simulink model "EV6_LUT_FourWheel_EV6Battery77p4kWh_PowerCorrected"  (R2024a)
settings: Solver=ode4  StartTime=0  StopTime=60  FixedStep=0.001  RelTol=1e-3
PreLoadFcn:
  | VSS_BICYCLE=Simulink.Variant('Dual=0');
  | VSS_DUAL=Simulink.Variant('Dual=1');
  | Dual=1;
  | load('DriveCycle2.mat')
PostLoadFcn:
  | if any(exist('dsrtsu_mdlpostloadfcn', 'file') ~= 0), dsrtsu_mdlpostloadfcn('Execute', bdroot); end
InitFcn:
  | , if any(exist('rtifpga_mdlclblib', 'file') ~= 0), rtifpga_mdlclblib('Init', bdroot); end,
  | , if any(exist('dsmpb_private', 'file') ~= 0), dsmpb_private('dsmpb_mdlclblib', 'Init', bdroot); end,
  | load('DriveCycle2.mat')
model workspace (MAT data in the model file):
  DiffRatio = 10.65
  EV6_2023_BattBranchCapacity_Ah = 55.5236728838
  EV6_2023_BattEnergy_kWh = 77.4
  EV6_2023_BattNominalVoltage_V = 697
  EV6_2023_BattNumCellsParallel = 2
  EV6_2023_BattNumCellsSeries = 192
  EV6_2023_BattOpenVoltCapBpts = [0 0.1 0.2 0.3 0.4 0.5 0.6 0.7 0.8 0.9 1]
  EV6_2023_BattOpenVoltTbl = [2.96762142548 3.40364281191 3.47417488548 3.54470541822 3.61523441014 3.68576186124 3.75628777151 3.82681214095 3.94527005036 4.07101207308 4.2120755254]
  EV6_2023_BattPackCapacity_Ah = 111.047345768
  EV6_2023_BattResistSocBpts = [0 0.2 0.4 0.6 0.8 1]
  EV6_2023_BattResistTbl = [0.0163620057716 0.0118174152018 0.00807187352333 0.00375663957972 0.00266904525531 0.00103635901355 0.0019014404175 0.0172368903217 0.0121226074867 0.00758541551769 0.00474065349228 0.00337561163613 ... (42 elements, 7x6)]
  EV6_2023_BattResistTempBpts = [243.1 253.1 263.1 273.1 283.1 298.1 313.1]
  EV6_2023_InitialPackOCV_V = 726.471714233
  EV6_2023_InitialSOC = 0.638878863672
  EV6_BattCellCapacity_Ah = 60.3
  EV6_BattInitialSOC = 0.638878863672
  EV6_BattOCV_Cell_V = [2.96762142548 3.40364281191 3.47417488548 3.54470541822 3.61523441014 3.68576186124 3.75628777151 3.82681214095 3.94527005036 4.07101207308 4.2120755254]
  EV6_BattOCV_SOC = [0 0.1 0.2 0.3 0.4 0.5 0.6 0.7 0.8 0.9 1]
  EV6_BattPackCapacity_Ah = 120.6
  EV6_BattParallelCells = 2
  EV6_BattResistanceSOC = [0 0.2 0.4 0.6 0.8 1]
  EV6_BattResistanceTable_Ohm = [0.0163620057716 0.0118174152018 0.00807187352333 0.00375663957972 0.00266904525531 0.00103635901355 0.0019014404175 0.0172368903217 0.0121226074867 0.00758541551769 0.00474065349228 0.00337561163613 ... (42 elements, 7x6)]
  EV6_BattResistanceTemp_K = [243.1 253.1 263.1 273.1 283.1 298.1 313.1]
  EV6_BattSeriesCells = 192
  EV6_FinalDriveRatio = 10.65
  EV6_TargetPackResistance_Ohm = 0.132763804608
  Gas = 0.383333333333
undefined symbols (not defined in the file): accel_bp_mps2, AccelCmd, ActTqLF_Nm_, ActTqLR_Nm_, ActTqRF_Nm_, ActTqRR_Nm_, BattChargeLimitMaxPwr, BattChargeLimitSocBpts, BattChargeLimitTbl, BattDischargeLimitSocBpts, BattDischargeLimitTbl, BattDischargeMaxPwr, BrakeMaxPrs, BrakeMaxTrq, ChassisDistCg2FrontAxle, ChassisDistCg2RearAxle, ChassisVehMass, CltchCmd, CoastDown, DecelCmd, DiscIntNeverNeededParam, EnvGravCnst, EnvPrs, EnvTemp, EV6_RegenTorqueGain, EV6_TractionTorqueGain, front_share_regen_3d, front_share_traction_3d, FuelSpecificGrav, GearCmd, h, InitStates, lgSw, limitedMCT, MCT, MtrEffSpdBpts, MtrEffTbl, MtrEffTrqBpts, MtrPwrMax, MtrTrqMax, out_1, pMCT, RealSimPara, Ref_speed, Ref_time, regen_torque_bp_Nm, speed_bp_kph, SteeringCmd, SupvsryCtrlRegenBrkCutOffTbl, SupvsryCtrlRegenSpdBpts, TestScnrioCycleNum, traction_torque_bp_Nm, US06, VEH
libraries: VSIGenLib x65, simulink x54, etargetslib x38, dsmpblib x24, vehdynlibtire x12, autolibshared x11, vehdynlibsuspension x7, vehdynlibtirecommon x7, autolibpowerinfoutils x6, autolibutils x5, autolibsharedcoupling x4, autolibmappedmotor x4
(part 13 of 19)

== system EV6_LUT_FourWheel_EV6Battery77p4kWh_PowerCorrected/Vehicle Under Test1/Vehicle/Vehicle Dynamics/Vehicle 14DOF/Suspension/MacPherson Front Suspension Solid Axle Rear Suspension/Vehicle Adapter ==
  Veh : Inport
  Bus Creator3 : BusCreator  Inputs=2
  Bus Selector1 : BusSelector  OutputSignals=InertFrm.FrntAxl.Lft.Disp.X,InertFrm.FrntAxl.Lft.Disp.Y,InertFrm.FrntAxl.Lft.Disp.Z,InertFrm.FrntAxl.Rght.Disp.X,InertFrm.FrntAxl.Rght.Disp.Y,InertFrm.FrntAxl.Rght.Disp.Z,InertFrm.RearAxl.Lft.Disp.X,InertFrm.RearAxl.Lft.Disp.Y,InertFrm.RearAxl.Lft.Disp.Z,InertFrm.RearAxl.Rght.Disp.X,InertFrm.RearAxl.Rght.Disp.Y,InertFrm.RearAxl.Rght.Disp.Z
  Bus Selector2 : BusSelector  OutputSignals=BdyFrm.FrntAxl.Lft.Vel.xdot,BdyFrm.FrntAxl.Lft.Vel.ydot,BdyFrm.FrntAxl.Lft.Vel.zdot,BdyFrm.FrntAxl.Rght.Vel.xdot,BdyFrm.FrntAxl.Rght.Vel.ydot,BdyFrm.FrntAxl.Rght.Vel.zdot,BdyFrm.RearAxl.Lft.Vel.xdot,BdyFrm.RearAxl.Lft.Vel.ydot,BdyFrm.RearAxl.Lft.Vel.zdot,BdyFrm.RearAxl.Rght.Vel.xdot,BdyFrm.RearAxl.Rght.Vel.ydot,BdyFrm.RearAxl.Rght.Vel.zdot
  Inertial Frame CG to Axle Offset : Constant  Value=[zeros(2,4);0.434 0.434 0.434 0.434]
  Mux1 : Mux  Inputs=12
  Mux2 : Mux  Inputs=12
  Reshape : Reshape  OutputDimensionality=Customize  OutputDimensions=[3,4]
  Reshape2 : Reshape  OutputDimensionality=Customize  OutputDimensions=[3,4]
  Scope{,1..3} (4 alike) : Scope
  Selector1 : Selector  NumberOfDimensions=2  InputPortWidth=3  IndexOptions=Index vector (dialog),Index vector (dialog)  Indices=[3],[1 2 3 4]  OutputSizes=1,1
  Selector13 : Selector  NumberOfDimensions=2  InputPortWidth=3  IndexOptions=Index vector (dialog),Index vector (dialog)  Indices=[3],[1 2 3 4]  OutputSizes=1,1
  Selector2 : Selector  NumberOfDimensions=2  InputPortWidth=3  IndexOptions=Index vector (dialog),Index vector (dialog)  Indices=[3],[1 2 3 4]  OutputSizes=1,1
  Sum : Sum  Inputs=|+-
  VehSusp : Outport  VectorParamsAs1DForOutWhenUnconnected=off
  wires:
  Sum/1 -> Selector1/1, Bus Creator3/1  "P"
  Inertial Frame CG to Axle Offset/1 -> Sum/2
  Mux2/1 -> Reshape/1
  Mux1/1 -> Reshape2/1
  Bus Selector2/12 -> Mux1/12  "<zdot>"
  Bus Selector2/11 -> Mux1/11  "<ydot>"
  Bus Selector2/10 -> Mux1/10  "<xdot>"
  Bus Selector2/9 -> Mux1/9  "<zdot>"
  Bus Selector2/8 -> Mux1/8  "<ydot>"
  Bus Selector2/7 -> Mux1/7  "<xdot>"
  Bus Selector2/6 -> Mux1/6  "<zdot>"
  Bus Selector2/5 -> Mux1/5  "<ydot>"
  Bus Selector2/4 -> Mux1/4  "<xdot>"
  Bus Selector2/3 -> Mux1/3  "<zdot>"
  Bus Selector2/2 -> Mux1/2  "<ydot>"
  Bus Selector2/1 -> Mux1/1  "<xdot>"
  Bus Selector1/12 -> Mux2/12  "<Z>"
  Bus Selector1/11 -> Mux2/11  "<Y>"
  Bus Selector1/10 -> Mux2/10  "<X>"
  Bus Selector1/9 -> Mux2/9  "<Z>"
  Bus Selector1/8 -> Mux2/8  "<Y>"
  Bus Selector1/7 -> Mux2/7  "<X>"
  Bus Selector1/6 -> Mux2/6  "<Z>"
  Bus Selector1/5 -> Mux2/5  "<Y>"
  Bus Selector1/4 -> Mux2/4  "<X>"
  Bus Selector1/3 -> Mux2/3  "<Z>"
  Bus Selector1/2 -> Mux2/2  "<Y>"
  Bus Selector1/1 -> Mux2/1  "<X>"
  Reshape/1 -> Scope2/1, Selector13/1, Sum/1
  Bus Creator3/1 -> VehSusp/1  "Veh"
  Reshape2/1 -> Selector2/1, Bus Creator3/2  "V"
  Veh/1 -> Bus Selector1/1, Bus Selector2/1
  Selector13/1 -> Scope/1
  Selector1/1 -> Scope1/1
  Selector2/1 -> Scope3/1

== system EV6_LUT_FourWheel_EV6Battery77p4kWh_PowerCorrected/Vehicle Under Test1/Vehicle/Vehicle Dynamics/Vehicle 14DOF/Suspension/MacPherson Front Suspension Solid Axle Rear Suspension/Wheel  Adapter ==
  Wheels : Inport
  Bus Selector : BusSelector  OutputSignals=TireFrame.Fx,TireFrame.Fy
  Bus Selector1 : BusSelector  OutputSignals=TireFrame.Re
  Bus Selector2 : BusSelector  OutputSignals=TireFrame.Mx,TireFrame.My,TireFrame.Mz
  Bus Selector3 : BusSelector  OutputSignals=TireFrame.z,TireFrame.zdot
  Matrix Concatenate : Concatenate  NumInputs=3  Mode=Multidimensional array
  Reshape{,1..7} (8 alike) : Reshape  OutputDimensionality=Row vector (2-D)
  Scope : Scope
  Scope1 : Scope
  Scope2 : Scope
  WhlFx : Outport  VectorParamsAs1DForOutWhenUnconnected=off
  WhlFy : Outport  Port=2  VectorParamsAs1DForOutWhenUnconnected=off
  z : Outport  Port=3  VectorParamsAs1DForOutWhenUnconnected=off
  zdot : Outport  Port=4  VectorParamsAs1DForOutWhenUnconnected=off
  M : Outport  Port=5  VectorParamsAs1DForOutWhenUnconnected=off
  Re : Outport  Port=6  VectorParamsAs1DForOutWhenUnconnected=off
  wires:
  Reshape/1 -> Scope1/1, z/1  "z"
  Matrix Concatenate/1 -> M/1  "M"
  Reshape5/1 -> Matrix Concatenate/3
  Reshape4/1 -> Matrix Concatenate/2
  Reshape3/1 -> Matrix Concatenate/1
  Bus Selector2/3 -> Reshape5/1  "<Mz>"
  Bus Selector2/2 -> Reshape4/1  "<My>"
  Bus Selector2/1 -> Reshape3/1  "<Mx>"
  Reshape1/1 -> Scope/1, Re/1  "Re"
  Bus Selector1/1 -> Reshape1/1  "<Re>"
  Reshape2/1 -> Scope2/1, zdot/1  "zdot"
  Bus Selector3/2 -> Reshape2/1  "<zdot>"
  Wheels/1 -> Bus Selector/1, Bus Selector3/1, Bus Selector2/1, Bus Selector1/1
  Bus Selector3/1 -> Reshape/1  "<z>"
  Bus Selector/2 -> Reshape7/1  "<Fy>"
  Bus Selector/1 -> Reshape6/1  "<Fx>"
  Reshape6/1 -> WhlFx/1
  Reshape7/1 -> WhlFy/1

== system EV6_LUT_FourWheel_EV6Battery77p4kWh_PowerCorrected/Vehicle Under Test1/Vehicle/Vehicle Dynamics/Vehicle 14DOF/Suspension/MacPherson Suspension/Steer Rate Adapter ==
  Veh : Inport
  Add : Sum
  Bus Selector3 : BusSelector  OutputSignals=BdyFrm.Cg.AngVel.r
  Constant : Constant  Value=zeros(1,4)
  Matrix Concatenate : Concatenate  NumInputs=3  Mode=Multidimensional array
  Matrix Concatenate1 : Concatenate  NumInputs=3  Mode=Multidimensional array
  Reshape2 : Reshape  OutputDimensionality=Row vector (2-D)
  Reshape3 : Reshape  OutputDimensionality=Row vector (2-D)
  Reshape4 : Reshape  OutputDimensionality=Row vector (2-D)
  Selector3 : Selector  InputPortWidth=1  IndexOptions=Index vector (dialog)  Indices=[1 1 1 1]  OutputSizes=1
  SteerRates : Constant  Value=zeros(1,4)
  AngVel : Outport  VectorParamsAs1DForOutWhenUnconnected=off
  wires:
  Add/1 -> AngVel/1  "AngVel"
  Veh/1 -> Bus Selector3/1
  Matrix Concatenate1/1 -> Add/1
  Reshape3/1 -> Matrix Concatenate/1, Matrix Concatenate/2
  Reshape4/1 -> Matrix Concatenate/3
  SteerRates/1 -> Reshape2/1
  Matrix Concatenate/1 -> Add/2
  Bus Selector3/1 -> Selector3/1  "<r>"
  Selector3/1 -> Reshape4/1
  Constant/1 -> Reshape3/1
  Reshape2/1 -> Matrix Concatenate1/2, Matrix Concatenate1/3, Matrix Concatenate1/1

== system EV6_LUT_FourWheel_EV6Battery77p4kWh_PowerCorrected/Vehicle Under Test1/Vehicle/Vehicle Dynamics/Vehicle 14DOF/Suspension/MacPherson Suspension/Steering Adapter ==
  Steer : Inport
  Reshape1 : Reshape  OutputDimensionality=Row vector (2-D)
  Selector : Selector  IndexOptions=Index vector (dialog)  Indices=[1 2]  OutputSizes=1
  StrgAng : Outport  VectorParamsAs1DForOutWhenUnconnected=off
  wires:
  Selector/1 -> Reshape1/1
  Steer/1 -> Selector/1
  Reshape1/1 -> StrgAng/1

== system EV6_LUT_FourWheel_EV6Battery77p4kWh_PowerCorrected/Vehicle Under Test1/Vehicle/Vehicle Dynamics/Vehicle 14DOF/Suspension/MacPherson Suspension/Vehicle Adapter ==
  Veh : Inport
  Bus Creator3 : BusCreator  Inputs=2
  Bus Selector1 : BusSelector  OutputSignals=InertFrm.FrntAxl.Lft.Disp.X,InertFrm.FrntAxl.Lft.Disp.Y,InertFrm.FrntAxl.Lft.Disp.Z,InertFrm.FrntAxl.Rght.Disp.X,InertFrm.FrntAxl.Rght.Disp.Y,InertFrm.FrntAxl.Rght.Disp.Z,InertFrm.RearAxl.Lft.Disp.X,InertFrm.RearAxl.Lft.Disp.Y,InertFrm.RearAxl.Lft.Disp.Z,InertFrm.RearAxl.Rght.Disp.X,InertFrm.RearAxl.Rght.Disp.Y,InertFrm.RearAxl.Rght.Disp.Z
  Bus Selector2 : BusSelector  OutputSignals=BdyFrm.FrntAxl.Lft.Vel.xdot,BdyFrm.FrntAxl.Lft.Vel.ydot,BdyFrm.FrntAxl.Lft.Vel.zdot,BdyFrm.FrntAxl.Rght.Vel.xdot,BdyFrm.FrntAxl.Rght.Vel.ydot,BdyFrm.FrntAxl.Rght.Vel.zdot,BdyFrm.RearAxl.Lft.Vel.xdot,BdyFrm.RearAxl.Lft.Vel.ydot,BdyFrm.RearAxl.Lft.Vel.zdot,BdyFrm.RearAxl.Rght.Vel.xdot,BdyFrm.RearAxl.Rght.Vel.ydot,BdyFrm.RearAxl.Rght.Vel.zdot
  Inertial Frame CG to Axle Offset : Constant  Value=[zeros(2,4);h*ones(1,4)]
  Mux1 : Mux  Inputs=12
  Mux2 : Mux  Inputs=12
  Reshape1 : Reshape  OutputDimensionality=Customize  OutputDimensions=[3,4]
  Reshape2 : Reshape  OutputDimensionality=Customize  OutputDimensions=[3,4]
  Sum : Sum  Inputs=|+-
  VehSusp : Outport  VectorParamsAs1DForOutWhenUnconnected=off
  wires:
  Reshape1/1 -> Sum/1
  Mux2/1 -> Reshape1/1
  Veh/1 -> Bus Selector1/1, Bus Selector2/1
  Sum/1 -> Bus Creator3/1  "P"
  Inertial Frame CG to Axle Offset/1 -> Sum/2
  Mux1/1 -> Reshape2/1
  Bus Selector2/12 -> Mux1/12  "<zdot>"
  Bus Selector2/11 -> Mux1/11  "<ydot>"
  Bus Selector2/10 -> Mux1/10  "<xdot>"
  Bus Selector2/9 -> Mux1/9  "<zdot>"
  Bus Selector2/8 -> Mux1/8  "<ydot>"
  Bus Selector2/7 -> Mux1/7  "<xdot>"
  Bus Selector2/6 -> Mux1/6  "<zdot>"
  Bus Selector2/5 -> Mux1/5  "<ydot>"
  Bus Selector2/4 -> Mux1/4  "<xdot>"
  Bus Selector2/3 -> Mux1/3  "<zdot>"
  Bus Selector2/2 -> Mux1/2  "<ydot>"
  Bus Selector2/1 -> Mux1/1  "<xdot>"
  Bus Selector1/12 -> Mux2/12  "<Z>"
  Bus Selector1/11 -> Mux2/11  "<Y>"
  Bus Selector1/10 -> Mux2/10  "<X>"
  Bus Selector1/9 -> Mux2/9  "<Z>"
  Bus Selector1/8 -> Mux2/8  "<Y>"
  Bus Selector1/7 -> Mux2/7  "<X>"
  Bus Selector1/6 -> Mux2/6  "<Z>"
  Bus Selector1/5 -> Mux2/5  "<Y>"
  Bus Selector1/4 -> Mux2/4  "<X>"
  Bus Selector1/3 -> Mux2/3  "<Z>"
  Bus Selector1/2 -> Mux2/2  "<Y>"
  Bus Selector1/1 -> Mux2/1  "<X>"
  Bus Creator3/1 -> VehSusp/1  "Veh"
  Reshape2/1 -> Bus Creator3/2  "V"

== system EV6_LUT_FourWheel_EV6Battery77p4kWh_PowerCorrected/Vehicle Under Test1/Vehicle/Vehicle Dynamics/Vehicle 14DOF/Suspension/MacPherson Suspension/Wheel  Adapter ==
  Wheels : Inport
  Bus Selector : BusSelector  OutputSignals=TireFrame.Fx,TireFrame.Fy
  Bus Selector1 : BusSelector  OutputSignals=TireFrame.Re
  Bus Selector2 : BusSelector  OutputSignals=TireFrame.Mx,TireFrame.My,TireFrame.Mz
  Bus Selector3 : BusSelector  OutputSignals=TireFrame.z,TireFrame.zdot
  Matrix Concatenate : Concatenate  NumInputs=3  Mode=Multidimensional array
  Reshape{,1..7} (8 alike) : Reshape  OutputDimensionality=Row vector (2-D)
  WhlFx : Outport  VectorParamsAs1DForOutWhenUnconnected=off
  WhlFy : Outport  Port=2  VectorParamsAs1DForOutWhenUnconnected=off
  z : Outport  Port=3  VectorParamsAs1DForOutWhenUnconnected=off
  zdot : Outport  Port=4  VectorParamsAs1DForOutWhenUnconnected=off
  M : Outport  Port=5  VectorParamsAs1DForOutWhenUnconnected=off
  Re : Outport  Port=6  VectorParamsAs1DForOutWhenUnconnected=off
  wires:
  Reshape/1 -> z/1  "z"
  Matrix Concatenate/1 -> M/1  "M"
  Reshape5/1 -> Matrix Concatenate/3
  Reshape4/1 -> Matrix Concatenate/2
  Reshape3/1 -> Matrix Concatenate/1
  Bus Selector2/3 -> Reshape5/1  "<Mz>"
  Bus Selector2/2 -> Reshape4/1  "<My>"
  Bus Selector2/1 -> Reshape3/1  "<Mx>"
  Reshape1/1 -> Re/1  "Re"
  Bus Selector1/1 -> Reshape1/1  "<Re>"
  Reshape2/1 -> zdot/1  "zdot"
  Bus Selector3/2 -> Reshape2/1  "<zdot>"
  Wheels/1 -> Bus Selector/1, Bus Selector3/1, Bus Selector2/1, Bus Selector1/1
  Bus Selector3/1 -> Reshape/1  "<z>"
  Bus Selector/2 -> Reshape7/1  "<Fy>"
  Bus Selector/1 -> Reshape6/1  "<Fx>"
  Reshape6/1 -> WhlFx/1
  Reshape7/1 -> WhlFy/1

== system EV6_LUT_FourWheel_EV6Battery77p4kWh_PowerCorrected/Vehicle Under Test1/Vehicle/Vehicle Dynamics/Vehicle 14DOF/Suspension/Mapped Suspension/Steer Rate Adapter ==
  Veh : Inport
  Add : Sum
  Bus Selector3 : BusSelector  OutputSignals=BdyFrm.Cg.AngVel.r
  Constant : Constant  Value=zeros(1,4)
  Matrix Concatenate : Concatenate  NumInputs=3  Mode=Multidimensional array
  Matrix Concatenate1 : Concatenate  NumInputs=3  Mode=Multidimensional array
  Reshape2 : Reshape  OutputDimensionality=Row vector (2-D)
  Reshape3 : Reshape  OutputDimensionality=Row vector (2-D)
  Reshape4 : Reshape  OutputDimensionality=Row vector (2-D)
  Selector3 : Selector  InputPortWidth=1  IndexOptions=Index vector (dialog)  Indices=[1 1 1 1]  OutputSizes=1
  SteerRates : Constant  Value=zeros(1,4)
  AngVel : Outport  VectorParamsAs1DForOutWhenUnconnected=off
  wires:
  Add/1 -> AngVel/1  "AngVel"
  Veh/1 -> Bus Selector3/1
  Matrix Concatenate1/1 -> Add/1
  Reshape3/1 -> Matrix Concatenate/1, Matrix Concatenate/2
  Reshape4/1 -> Matrix Concatenate/3
  SteerRates/1 -> Reshape2/1
  Matrix Concatenate/1 -> Add/2
  Bus Selector3/1 -> Selector3/1  "<r>"
  Selector3/1 -> Reshape4/1
  Constant/1 -> Reshape3/1
  Reshape2/1 -> Matrix Concatenate1/2, Matrix Concatenate1/3, Matrix Concatenate1/1

== system EV6_LUT_FourWheel_EV6Battery77p4kWh_PowerCorrected/Vehicle Under Test1/Vehicle/Vehicle Dynamics/Vehicle 14DOF/Suspension/Mapped Suspension/Vehicle Adapter ==
  Veh : Inport
  Bus Creator3 : BusCreator  Inputs=2
  Bus Selector1 : BusSelector  OutputSignals=InertFrm.FrntAxl.Lft.Disp.X,InertFrm.FrntAxl.Lft.Disp.Y,InertFrm.FrntAxl.Lft.Disp.Z,InertFrm.FrntAxl.Rght.Disp.X,InertFrm.FrntAxl.Rght.Disp.Y,InertFrm.FrntAxl.Rght.Disp.Z,InertFrm.RearAxl.Lft.Disp.X,InertFrm.RearAxl.Lft.Disp.Y,InertFrm.RearAxl.Lft.Disp.Z,InertFrm.RearAxl.Rght.Disp.X,InertFrm.RearAxl.Rght.Disp.Y,InertFrm.RearAxl.Rght.Disp.Z
  Bus Selector2 : BusSelector  OutputSignals=BdyFrm.FrntAxl.Lft.Vel.xdot,BdyFrm.FrntAxl.Lft.Vel.ydot,BdyFrm.FrntAxl.Lft.Vel.zdot,BdyFrm.FrntAxl.Rght.Vel.xdot,BdyFrm.FrntAxl.Rght.Vel.ydot,BdyFrm.FrntAxl.Rght.Vel.zdot,BdyFrm.RearAxl.Lft.Vel.xdot,BdyFrm.RearAxl.Lft.Vel.ydot,BdyFrm.RearAxl.Lft.Vel.zdot,BdyFrm.RearAxl.Rght.Vel.xdot,BdyFrm.RearAxl.Rght.Vel.ydot,BdyFrm.RearAxl.Rght.Vel.zdot
  Inertial Frame CG to Axle Offset : Constant  Value=[zeros(2,4);h*ones(1,4)]
  Mux1 : Mux  Inputs=12
  Mux2 : Mux  Inputs=12
  Reshape : Reshape  OutputDimensionality=Customize  OutputDimensions=[3,4]
  Reshape2 : Reshape  OutputDimensionality=Customize  OutputDimensions=[3,4]
  Sum : Sum  Inputs=|+-
  VehSusp : Outport  VectorParamsAs1DForOutWhenUnconnected=off
  wires:
  Sum/1 -> Bus Creator3/1  "P"
  Inertial Frame CG to Axle Offset/1 -> Sum/2
  Mux2/1 -> Reshape/1
  Mux1/1 -> Reshape2/1
  Bus Selector2/12 -> Mux1/12  "<zdot>"
  Bus Selector2/11 -> Mux1/11  "<ydot>"
  Bus Selector2/10 -> Mux1/10  "<xdot>"
  Bus Selector2/9 -> Mux1/9  "<zdot>"
  Bus Selector2/8 -> Mux1/8  "<ydot>"
  Bus Selector2/7 -> Mux1/7  "<xdot>"
  Bus Selector2/6 -> Mux1/6  "<zdot>"
  Bus Selector2/5 -> Mux1/5  "<ydot>"
  Bus Selector2/4 -> Mux1/4  "<xdot>"
  Bus Selector2/3 -> Mux1/3  "<zdot>"
  Bus Selector2/2 -> Mux1/2  "<ydot>"
  Bus Selector2/1 -> Mux1/1  "<xdot>"
  Bus Selector1/12 -> Mux2/12  "<Z>"
  Bus Selector1/11 -> Mux2/11  "<Y>"
  Bus Selector1/10 -> Mux2/10  "<X>"
  Bus Selector1/9 -> Mux2/9  "<Z>"
  Bus Selector1/8 -> Mux2/8  "<Y>"
  Bus Selector1/7 -> Mux2/7  "<X>"
  Bus Selector1/6 -> Mux2/6  "<Z>"
  Bus Selector1/5 -> Mux2/5  "<Y>"
  Bus Selector1/4 -> Mux2/4  "<X>"
  Bus Selector1/3 -> Mux2/3  "<Z>"
  Bus Selector1/2 -> Mux2/2  "<Y>"
  Bus Selector1/1 -> Mux2/1  "<X>"
  Reshape/1 -> Sum/1
  Bus Creator3/1 -> VehSusp/1  "Veh"
  Reshape2/1 -> Bus Creator3/2  "V"
  Veh/1 -> Bus Selector1/1, Bus Selector2/1

== system EV6_LUT_FourWheel_EV6Battery77p4kWh_PowerCorrected/Vehicle Under Test1/Vehicle/Vehicle Dynamics/Vehicle 14DOF/Suspension/Mapped Suspension/Wheel  Adapter ==
  Wheels : Inport
  Bus Selector : BusSelector  OutputSignals=TireFrame.Fx,TireFrame.Fy
  Bus Selector1 : BusSelector  OutputSignals=TireFrame.Re
  Bus Selector2 : BusSelector  OutputSignals=TireFrame.Mx,TireFrame.My,TireFrame.Mz
  Bus Selector3 : BusSelector  OutputSignals=TireFrame.z,TireFrame.zdot
  Matrix Concatenate : Concatenate  NumInputs=3  Mode=Multidimensional array
  Reshape{,1..7} (8 alike) : Reshape  OutputDimensionality=Row vector (2-D)
  WhlFx : Outport  VectorParamsAs1DForOutWhenUnconnected=off
  WhlFy : Outport  Port=2  VectorParamsAs1DForOutWhenUnconnected=off
  z : Outport  Port=3  VectorParamsAs1DForOutWhenUnconnected=off
  zdot : Outport  Port=4  VectorParamsAs1DForOutWhenUnconnected=off
  M : Outport  Port=5  VectorParamsAs1DForOutWhenUnconnected=off
  Re : Outport  Port=6  VectorParamsAs1DForOutWhenUnconnected=off
  wires:
  Reshape/1 -> z/1  "z"
  Matrix Concatenate/1 -> M/1  "M"
  Reshape5/1 -> Matrix Concatenate/3
  Reshape4/1 -> Matrix Concatenate/2
  Reshape3/1 -> Matrix Concatenate/1
  Bus Selector2/3 -> Reshape5/1  "<Mz>"
  Bus Selector2/2 -> Reshape4/1  "<My>"
  Bus Selector2/1 -> Reshape3/1  "<Mx>"
  Reshape1/1 -> Re/1  "Re"
  Bus Selector1/1 -> Reshape1/1  "<Re>"
  Reshape2/1 -> zdot/1  "zdot"
  Bus Selector3/2 -> Reshape2/1  "<zdot>"
  Wheels/1 -> Bus Selector/1, Bus Selector3/1, Bus Selector2/1, Bus Selector1/1
  Bus Selector3/1 -> Reshape/1  "<z>"
  Bus Selector/2 -> Reshape7/1  "<Fy>"
  Bus Selector/1 -> Reshape6/1  "<Fx>"
  Reshape6/1 -> WhlFx/1
  Reshape7/1 -> WhlFy/1

== system EV6_LUT_FourWheel_EV6Battery77p4kWh_PowerCorrected/Vehicle Under Test1/Vehicle/Vehicle Dynamics/Vehicle 14DOF/Vehicle/Variant Subsystem/3DOF ==
  Suspension : Inport
  Wind : Inport  Port=2
  Bus Selector1 : BusSelector  OutputSignals=Veh.F
  Permute Dimensions : PermuteDimensions
  Permute Dimensions1 : PermuteDimensions
  Scope : Scope
  Scope1 : Scope  NumInputPorts=2
  Scope2 : Scope  NumInputPorts=2
  Scope3 : Scope
  Scope4 : Scope
  Selector : Selector  NumberOfDimensions=2  InputPortWidth=3  IndexOptions=Index vector (dialog),Index vector (dialog)  Indices=[1 2],[1 2]  OutputSizes=1,1
  Selector1 : Selector  NumberOfDimensions=2  InputPortWidth=3  IndexOptions=Index vector (dialog),Index vector (dialog)  Indices=[1 2],[3 4]  OutputSizes=1,1
  Signal Specification : SignalSpecification  Unit=N
  Signal Specification1 : SignalSpecification  Unit=N
  Terminator{,1..5} (6 alike) : Terminator
  Vehicle Body 3DOF Dual Track : autolibshared/Vehicle Body 3DOF Single Track  trackMode=Dual  inputMode=External forces  frontSteerMode=off  rearSteerMode=off  windMode=on  muMode=off  extFMode=off  extMMode=off  htchFMode=off  htchMMode=off  extXo=off  extpsio=off  extxdoto=off  extro=off  extYo=off  extTamb=off  extydoto=off  aMode=2  NF=2  NR=2  m=2040  a=1.4  b=1.6  h=0.5  dh=1  hh=0.2  X_o=0  xdot_o=0  CalphaMode=off  sigmaMode=on  d=0  hl=0  w=1.9.*[1 1]  Cy_f=12e3  Cy_r=11e3  sigma_f=.1  sigma_r=.1  alpha_f_brk=[-.1 .1]  Cy_f_data=[-9e3 9e3]  alpha_r_brk=[-.1 .1]  Cy_r_data=[-9e3 9e3]  Y_o=0  ydot_o=0  Izz=2100  psi_o=0  r_o=0  Af=2  Cd=.3  Cl=.1  Cpm=.1  beta_w=[0:0.001:0.01]  Cs=[0:0.01:0.1]  Cym=[0:0.001:0.01]  Pabs=101325  Tair=273  g=9.81  mu=1  xdot_tol=.1  Fznom=5000  Fxtire_sat=7e5  Fytire_sat=7e5  longOff=0  latOff=0  vertOff=0  wrapAng=on
  VehFdbk : Outport  VectorParamsAs1DForOutWhenUnconnected=off
  wires:
  Wind/1 -> Vehicle Body 3DOF Dual Track/3
  Permute Dimensions/1 -> Signal Specification1/1
  Permute Dimensions1/1 -> Signal Specification/1
  Vehicle Body 3DOF Dual Track/7 -> Terminator5/1, Scope1/2
  Vehicle Body 3DOF Dual Track/1 -> VehFdbk/1
  Vehicle Body 3DOF Dual Track/2 -> Terminator/1, Scope/1
  Vehicle Body 3DOF Dual Track/4 -> Terminator2/1
  Vehicle Body 3DOF Dual Track/6 -> Terminator4/1, Scope1/1
  Signal Specification/1 -> Scope4/1, Vehicle Body 3DOF Dual Track/2
  Vehicle Body 3DOF Dual Track/3 -> Terminator1/1
  Signal Specification1/1 -> Vehicle Body 3DOF Dual Track/1, Scope3/1
  Vehicle Body 3DOF Dual Track/5 -> Terminator3/1
  Suspension/1 -> Bus Selector1/1
  Selector1/1 -> Permute Dimensions1/1
  Selector/1 -> Permute Dimensions/1
  Bus Selector1/1 -> Selector/1, Selector1/1  "<F>"

== system EV6_LUT_FourWheel_EV6Battery77p4kWh_PowerCorrected/Vehicle Under Test1/Vehicle/Vehicle Dynamics/Vehicle 14DOF/Vehicle/Variant Subsystem/6DOF ==
  Suspension : Inport
  Wind : Inport  Port=2
  Bus Selector3 : BusSelector  OutputSignals=Veh.F,Veh.M
  Constant : Constant  Value=[0;0;0]
  Constant1 : Constant  Value=[0;0;0]
  Terminator{,1..5} (6 alike) : Terminator
  Vehicle Body 6DOF : vehdynlibeom/Vehicle Body 6DOF  extPos=on  extVel=on  extEuler=on  extRotRate=on  htchFMode=off  htchMMode=off  m=2040  a=1.4  b=1.6  d=0  h=0.5  dh=1  hl=0  hh=0.1  Xe_o=[0,0,0.1]  xbdot_o=[0,0,0]  eul_o=[0,0,0]  p_o=[0,0,0]  Iveh=[430 0 0; 0 1900 0; 0 0 2100]  w=[1.9,1.9]  z1m=0  z1R=[-.25,.125,.15]  z1I=[1.4,-.2,.1;-.2,1.4,.1;.1,.1,2.25].*0  z2m=0  z2R=[1.4,0,.8]  z2I=[1.4,-.2,.1;-.2,1.4,.1;.1,.1,2.25].*0  z3m=0  z3R=[.75,-.5,.4]  z3I=[5,-.1,-2;-2,9,.1;-.1,.1,6].*0  z4m=0  z4R=[.75,.5,.4]  z4I=[5,-.1,-2;-2,9,.1;-.1,.1,6].*0  z5m=0  z5R=[1.25,-.5,.4]  z5I=[5,-.1,-2;-2,9,.1;-.1,.1,6].*0  z6m=0  z6R=[1.25,-.5,.4]  z6I=[5,-.1,-2;-2,9,.1;-.1,.1,6].*0  z7m=0  z7R=[2,0,.25]  z7I=[1.4,-.2,.1;-.2,1.4,.1;.1,.1,2.25].*0  Af=2  Cd=.3  Cl=.1  Cpm=.1  beta_w=[0:0.001:0.01]  Cs=[0:0.01:0.1]  Cym=[0:0.001:0.01]  Pabs=101325  extTamb=off  Tair=273  g=9.81  xdot_tol=.1  longOff=0  latOff=0  vertOff=0  wrapAng=on  aMode=2
  VehFdbk : Outport  VectorParamsAs1DForOutWhenUnconnected=off
  wires:
  Vehicle Body 6DOF/7 -> Terminator5/1
  Vehicle Body 6DOF/6 -> Terminator4/1
  Vehicle Body 6DOF/5 -> Terminator3/1
  Vehicle Body 6DOF/4 -> Terminator2/1
  Vehicle Body 6DOF/3 -> Terminator1/1
  Vehicle Body 6DOF/2 -> Terminator/1
  Constant1/1 -> Vehicle Body 6DOF/4
  Vehicle Body 6DOF/1 -> VehFdbk/1  "VehFdbk"
  Suspension/1 -> Bus Selector3/1
  Constant/1 -> Vehicle Body 6DOF/3
  Wind/1 -> Vehicle Body 6DOF/5
  Bus Selector3/1 -> Vehicle Body 6DOF/1  "<F>"
  Bus Selector3/2 -> Vehicle Body 6DOF/2  "<M>"

== system EV6_LUT_FourWheel_EV6Battery77p4kWh_PowerCorrected/Vehicle Under Test1/Vehicle/Vehicle Dynamics/Vehicle 14DOF/Wheels and Tires/VDBS/Tire2Veh ==
  Wheel : Inport
  Fz : Inport  Port=2
  WheelCamber : Inport  Port=3
  WheelSteer : Inport  Port=4
  Bus Creator : BusCreator  Inputs=2
  Bus Creator1 : BusCreator  Inputs=2
  Bus Selector7 : BusSelector  OutputSignals=Omega,Fx,Fy,Mz,Mx,My,Re,z,zdot,Kappa,Alpha
  Dead Zone2 : DeadZone  LowerValue=-5  UpperValue=5  ZeroCross=off
  Dead Zone3 : DeadZone  LowerValue=-10  UpperValue=10  ZeroCross=off
  Demux : Demux  Outputs=[2,2]
  Demux1 : Demux  Outputs=[2,2]
  Math Function : Math  Operator=transpose  SignedPower=on
  Reshape6 : Reshape  OutputDimensionality=Customize  OutputDimensions=[2,2]
  Routiong : Subsystem
  Vector Concatenate5 : Concatenate  Mode=Multidimensional array  ConcatenateDimension=2
  Vector Concatenate6 : Concatenate  Mode=Multidimensional array  ConcatenateDimension=2
  Vector Concatenate8 : Concatenate  NumInputs=3  Mode=Multidimensional array  ConcatenateDimension=2
  Wheel Angles : Subsystem
  Wheel to Body Transform : Subsystem
  Wheels : Outport  VectorParamsAs1DForOutWhenUnconnected=off
  Omega : Outport  Port=2  VectorParamsAs1DForOutWhenUnconnected=off
  FrntAxlF : Outport  Port=3  VectorParamsAs1DForOutWhenUnconnected=off
  RearAxlF : Outport  Port=4  VectorParamsAs1DForOutWhenUnconnected=off
  <Mz> : Outport  Port=5  VectorParamsAs1DForOutWhenUnconnected=off
  SuspWhlPz : Outport  Port=6  VectorParamsAs1DForOutWhenUnconnected=off
  SuspWhlVz : Outport  Port=7  VectorParamsAs1DForOutWhenUnconnected=off
  wires:
  Bus Selector7/11 -> Routiong/8(<Alpha>)  "<Alpha>"
  Bus Creator/1 -> Bus Creator1/2  "Steering"
  [CamberAngles] -> Bus Creator/2  "Camber Angles"
  Routiong/1(Out1) -> Bus Creator1/1  "TireFrame"
  Bus Creator1/1 -> Wheels/1  "Wheels"
  [WheelAngles] -> Bus Creator/1  "Wheel Angles"
  Routiong/3(Out3) -> SuspWhlVz/1
  Routiong/2(Out2) -> SuspWhlPz/1
  Bus Selector7/10 -> Routiong/7(<Kappa>)  "<Kappa>"
  Bus Selector7/9 -> Routiong/6(<zdot>)  "<zdot>"
  [Fz] -> Routiong/12(Fz)  "Fz"
  [Fy] -> Routiong/11(Fy)  "Fy"
  Bus Selector7/8 -> Routiong/5(<z>)  "<z>"
  [Fx] -> Routiong/10(Fx)  "Fx"
  [omega] -> Routiong/9(Omega)  "omega"
  Bus Selector7/7 -> Routiong/4(<Re>)  "<Re>"
  Bus Selector7/6 -> Routiong/3(<My>)  "<My>"
  Bus Selector7/5 -> Routiong/2(<Mx>)  "<Mx>"
  Bus Selector7/3 -> Dead Zone3/1  "<Fy>"
  WheelCamber/1 -> [CamberAngles], Wheel Angles/2(Camber)
  Wheel to Body Transform/3(Fz) -> [Fz]
  Bus Selector7/4 -> Routiong/1(<Mz>), <Mz>/1  "<Mz>"
  WheelSteer/1 -> [WheelAngles], Wheel Angles/1(Front)
  Bus Selector7/1 -> Reshape6/1, [omega]  "<Omega>"
  Wheel Angles/1(Vehicle) -> Wheel to Body Transform/2(WheelAngles)
  Wheel to Body Transform/2(Fy) -> [Fy], Demux1/1  "Fy"
  Demux1/1 -> Vector Concatenate5/2
  Reshape6/1 -> Omega/1
  Wheel/1 -> Bus Selector7/1
  Vector Concatenate5/1 -> FrntAxlF/1
  Wheel to Body Transform/1(Fx) -> Demux/1, [Fx]  "Fx"
  Dead Zone2/1 -> Vector Concatenate8/1
  Bus Selector7/2 -> Dead Zone2/1  "<Fx>"
  Dead Zone3/1 -> Vector Concatenate8/2
  Math Function/1 -> Wheel to Body Transform/1(Forces)
  Demux/1 -> Vector Concatenate5/1
  Demux1/2 -> Vector Concatenate6/2
  Demux/2 -> Vector Concatenate6/1
  Vector Concatenate8/1 -> Math Function/1
  Vector Concatenate6/1 -> RearAxlF/1
  Fz/1 -> Vector Concatenate8/3

== system EV6_LUT_FourWheel_EV6Battery77p4kWh_PowerCorrected/Vehicle Under Test1/Vehicle/Vehicle Dynamics/Vehicle 14DOF/Wheels and Tires/VDBS/Tires ==
  "DriveTorque " : Inport
  "Brake Pressure " : Inport  Port=2
  "r " : Inport  Port=3
  "Vx " : Inport  Port=4
  "Vy " : Inport  Port=5
  "Camber " : Inport  Port=6
  "Press " : Inport  Port=7
  "lambda " : Inport  Port=8
  "Gnd " : Inport  Port=9
  "FzSusp " : Inport  Port=10
  Fiala Tires : Subsystem  VariantControl=1
  MF Tires : Subsystem  VariantControl=0
  " Wheels" : Outport  VectorParamsAs1DForOutWhenUnconnected=off

== system EV6_LUT_FourWheel_EV6Battery77p4kWh_PowerCorrected/Vehicle Under Test1/Vehicle/Vehicle Dynamics/Vehicle 14DOF/Wheels and Tires/VDBS/Veh2Tire ==
  r : Inport
  Axle : Inport  Port=2
  Brake : Inport  Port=3
  VehVel : Inport  Port=4
  WheelSteer : Inport  Port=5
  WheelCamber : Inport  Port=6
  Demux4 : Demux
  Gain4 : Gain  Gain=[1;-1;1;-1]*0+1
  Mux1 : Mux
  Reshape3 : Reshape
  Reshape4 : Reshape
  Unary Minus : UnaryMinus
  Wheel Angles : Subsystem
  Wheel to Body Transform : Subsystem
  T : Outport  Unit=N*m  VectorParamsAs1DForOutWhenUnconnected=off
  P : Outport  Port=2  Unit=Pa  VectorParamsAs1DForOutWhenUnconnected=off
  psidot : Outport  Port=3  Unit=rad/s  VectorParamsAs1DForOutWhenUnconnected=off
  xdotAxle : Outport  Port=4  Unit=m/s  VectorParamsAs1DForOutWhenUnconnected=off
  ydotAxle : Outport  Port=5  Unit=m/s  VectorParamsAs1DForOutWhenUnconnected=off
  zdotAxle : Outport  Port=6  Unit=m/s  VectorParamsAs1DForOutWhenUnconnected=off
  wires:
  Wheel Angles/1(Vehicle) -> Wheel to Body Transform/2(WheelAngles)
  Unary Minus/1 -> psidot/1
  WheelCamber/1 -> Wheel Angles/2(camber)
  Wheel to Body Transform/3(zdotWheel) -> zdotAxle/1  "Vz"
  VehVel/1 -> Wheel to Body Transform/1(VelVeh)
  Reshape4/1 -> Gain4/1
  Gain4/1 -> T/1
  Reshape3/1 -> Demux4/1
  Demux4/3 -> Mux1/3
  r/1 -> Unary Minus/1
  Mux1/1 -> P/1
  WheelSteer/1 -> Wheel Angles/1(steer)
  Wheel to Body Transform/2(ydotWheel) -> ydotAxle/1  "Vy"
  Demux4/2 -> Mux1/2
  Wheel to Body Transform/1(xdotWheel) -> xdotAxle/1  "Vx"
  Axle/1 -> Reshape4/1
  Demux4/4 -> Mux1/4
  Brake/1 -> Reshape3/1
  Demux4/1 -> Mux1/1

== system EV6_LUT_FourWheel_EV6Battery77p4kWh_PowerCorrected/Vehicle Under Test1/Vehicle/Vehicle Dynamics/Vehicle 14DOF/Wheels and Tires/VDBS/scale factors with friction ==
  lamda_mu_x : Inport
  lamda_mu_y : Inport  Port=2
  0 : Constant  Value=[zeros(1,numWheels)]  VectorParams1D=off
  Reshape : Reshape  OutputDimensionality=Row vector (2-D)  OutputDimensions=[1,numWheels]
  Reshape1 : Reshape  OutputDimensionality=Row vector (2-D)  OutputDimensions=[1,numWheels]
  Signal Specification3 : SignalSpecification  Unit=1
  Vector Concatenate : Concatenate  NumInputs=5  Mode=Multidimensional array
  ones : Constant  Value=[ones(23,numWheels)]  VectorParams1D=off
  ones2 : Constant  Value=ones(1,numWheels)  VectorParams1D=off
  lambdas : Outport  Unit=1  VectorParamsAs1DForOutWhenUnconnected=off
  wires:
  Signal Specification3/1 -> lambdas/1
  Reshape/1 -> Vector Concatenate/2
  Reshape1/1 -> Vector Concatenate/3
  0/1 -> Vector Concatenate/4  "lamda_mu_V"
  ones/1 -> Vector Concatenate/5
  Vector Concatenate/1 -> Signal Specification3/1
  ones2/1 -> Vector Concatenate/1  "lambda_Fz0"
  lamda_mu_x/1 -> Reshape/1
  lamda_mu_y/1 -> Reshape1/1

== system EV6_LUT_FourWheel_EV6Battery77p4kWh_PowerCorrected/Vehicle Under Test1/Vehicle/Vehicle Dynamics/Vehicle 7DOF/Longitudinal Wheels 4DOF/Axle Forces/Bicycle ==
  F : Inport
  R : Inport  Port=2
  Sum of Elements : Sum  Inputs=+
  Sum of Elements1 : Sum  Inputs=+
  FrntAxlF : Outport  Unit=N  VectorParamsAs1DForOutWhenUnconnected=off
  RearAxlF : Outport  Port=2  Unit=N  VectorParamsAs1DForOutWhenUnconnected=off
  wires:
  F/1 -> Sum of Elements/1
  R/1 -> Sum of Elements1/1
  Sum of Elements1/1 -> RearAxlF/1
  Sum of Elements/1 -> FrntAxlF/1

== system EV6_LUT_FourWheel_EV6Battery77p4kWh_PowerCorrected/Vehicle Under Test1/Vehicle/Vehicle Dynamics/Vehicle 7DOF/Longitudinal Wheels 4DOF/Axle Forces/Dual ==
  F : Inport
  R : Inport  Port=2
  FrntAxlF : Outport  Unit=N  VectorParamsAs1DForOutWhenUnconnected=off
  RearAxlF : Outport  Port=2  Unit=N  VectorParamsAs1DForOutWhenUnconnected=off
  wires:
  F/1 -> FrntAxlF/1
  R/1 -> RearAxlF/1

== system EV6_LUT_FourWheel_EV6Battery77p4kWh_PowerCorrected/Vehicle Under Test1/Vehicle/Vehicle Dynamics/Vehicle 7DOF/Longitudinal Wheels 4DOF/Tires/4-by-1 Gnd ==
  Constant : Constant  Value=0
  Vector Concatenate : Concatenate  NumInputs=4
  Gnd : Outport
  wires:
  Vector Concatenate/1 -> Gnd/1
  Constant/1 -> Vector Concatenate/1, Vector Concatenate/2, Vector Concatenate/3, Vector Concatenate/4

== system EV6_LUT_FourWheel_EV6Battery77p4kWh_PowerCorrected/Vehicle Under Test1/Vehicle/Vehicle Dynamics/Vehicle 7DOF/Longitudinal Wheels 4DOF/Tires/4-by-1 Gnd1 ==
  Constant : Constant  Value=0
  Vector Concatenate : Concatenate  NumInputs=4
  Gnd : Outport
  wires:
  Vector Concatenate/1 -> Gnd/1
  Constant/1 -> Vector Concatenate/1, Vector Concatenate/2, Vector Concatenate/3, Vector Concatenate/4

== system EV6_LUT_FourWheel_EV6Battery77p4kWh_PowerCorrected/Vehicle Under Test1/Vehicle/Vehicle Dynamics/Vehicle 7DOF/Longitudinal Wheels 4DOF/Tires/4-by-1 Gnd2 ==
  Constant : Constant  Value=0
  Vector Concatenate : Concatenate  NumInputs=4
  Gnd : Outport
  wires:
  Vector Concatenate/1 -> Gnd/1
  Constant/1 -> Vector Concatenate/1, Vector Concatenate/2, Vector Concatenate/3, Vector Concatenate/4

== system EV6_LUT_FourWheel_EV6Battery77p4kWh_PowerCorrected/Vehicle Under Test1/Vehicle/Vehicle Dynamics/Vehicle 7DOF/Longitudinal Wheels 4DOF/Tires/4-by-1 Gnd3 ==
  Constant : Constant  Value=0
  Vector Concatenate : Concatenate  NumInputs=4
  Gnd : Outport
  wires:
  Vector Concatenate/1 -> Gnd/1
  Constant/1 -> Vector Concatenate/1, Vector Concatenate/2, Vector Concatenate/3, Vector Concatenate/4
